simulink model "pwtsimplificado_longitudinal"  (R2025a)
settings: Solver=ode3  StartTime=0.0  StopTime=12  FixedStep=Amostragem/10  RelTol=1e-3
InitFcn:
  | % Suprime os warnings de limite do MFeval. Eles disparam A CADA PASSO quando o pneu
  | % opera fora da faixa do .tir (frenagem forte, baixa velocidade, Fz baixo) e chegam a
  | % custar 10x o tempo de simulacao. Os valores ja sao saturados internamente pelo solver.
  | warning('off','Solver:Limits:Exceeded');
  | warning('off','Solver:CoeffChecks:Ex');
model workspace (MATLAB code in the model file):
  | %% =======================================================================
  | %  INICIALIZACAO - Powertrain VE (motor de inducao Hercules AMP223/226
  | %  + SEVCON Gen5, IRFOC)  -  rev. 4 (identificacao + fix Vmag + dados AMP-226)
  | %  -----------------------------------------------------------------------
  | %  CONVENCAO: correntes/tensoes de fase em VALORES DE PICO (Park/Clarke
  | %  amplitude-invariantes). Valores RMS da folha convertidos com sqrt(2).
  | %
  | %  PARAMETROS DO MOTOR: identificados por minimos quadrados sobre as 20
  | %  linhas das tabelas do dinamometro (residuo RMS 3.3%). Modelo LINEAR,
  | %  valido na regiao de fluxo parcial (Id <= ~110 A pico) onde o modelo e
  | %  o controlador operam. Os valores de placa "133 A nominal" e "114 A a
  | %  vazio" sao pontos de fluxo pleno SATURADO - o modelo linear NAO os
  | %  reproduz e NAO deve reproduzir. NAO "corrigir" Imag de volta p/ 114*sqrt(2).
  | %
  | %  ATENCAO: o BLOCO DA MAQUINA no subsistema Motor precisa carregar estes
  | %  mesmos Lm/Lls/Llr/Rr/Rs - controlador e planta com motores diferentes
  | %  recria o descasamento que ja foi depurado.
  | %% =======================================================================
  | %% --- Acumulador (lado DC) ----------------------------------------------
  | Bi = 250 ;             % Corrente DC maxima do acumulador (A) - limite de POTENCIA no lado DC.
  |                        %   NAO usar como limite de corrente de fase (ver I_max).
  |                        %   Com 28 kW de pico e EFF ~83%: 234 A @144V -> so 6% de folga.
  | Bv = 168 ;             % Tensao do acumulador (V) - carga cheia (nominal ~144 V)
  | %% --- Motor (identificado a partir das tabelas da folha) ----------------
  | Pnom  = 11000 ;        % Potencia nominal do motor (W)
  | T_max = 94 ;           % Torque maximo/pico 2-min (N*m) - usar na saturacao de Torque_ref
  | Poles = 2 ;            % Numero de PARES de polos (motor de 4 polos -> Poles = 2)
  | Rs  = 0.0165 ;         % Resistencia do estator por fase (Ohm) - folha obs.9: 0.033 de linha /2
  |                        %   (a identificacao usou 0.0144 fixo; diferenca so mexe ~7% no Ki)
  | Rr  = 0.01858 ;        % Resistencia do rotor referida ao estator (Ohm) - IDENTIFICADO
  |                        %   NUNCA usar 0.0248/0.0139: 0.0248 veio do Tau_r=35.5ms
  |                        %   INTERMEDIARIO ERRADO (assumia Kt/Imag antigos); reverter se aparecer.
  | Lls = 7.4763e-5 ;      % Indutancia de dispersao do estator (H) - IDENTIFICADO (Lls=Llr imposto)
  | Llr = 7.4763e-5 ;      % Indutancia de dispersao do rotor (H)   - IDENTIFICADO
  | Lm  = 1.0357e-3 ;      % Indutancia de magnetizacao (H) - IDENTIFICADO (valor LINEAR, fluxo parcial)
  | Ls  = Lls + Lm ;       % Indutancia total do estator (H)  = 1.1105e-3
  | Lr  = Lm + Llr ;       % Indutancia total do rotor (H)    = 1.1105e-3
  | Im  = 0.0071 ;         % Inercia do rotor (kg*m^2). A folha escreve "kgfm2" mas o valor e SI:
  |                        %   carcaca 100 limita o rotor a r<~7cm -> J~0.007-0.01 kg*m^2;
  |                        %   0.0697 (x9.81) exigiria r~12cm, impossivel. [dica: Im=100 trava o rotor]
  | motor_eff = 0.874 ;    % Eficiencia nominal do motor (-) (folha: 87.4% nominal, ~83% no pico)
  | mc_eff    = 0.95 ;     % Eficiencia do inversor (-)
  | %% --- Constantes derivadas do motor -------------------------------------
  | sigma = 1 - (Lm^2)/(Ls*Lr) ;      % Coef. de dispersao total (-)             ~0.1301
  | Tau_r = Lr/Rr ;                   % Constante de tempo do rotor (s)          ~59.8 ms
  |                                   %   Gain "1/Tau_r" embutido no modelo -> 16.73
  | Kt    = (3/2)*Poles*(Lm^2/Lr) ;   % Constante de torque p/ correntes de PICO ~2.898e-3 N*m/A^2
  | Req   = Rs + Rr*((Lm/Lr)^2) ;     % Resistencia equivalente da malha de corrente (Ohm) ~0.0327
  | %% --- Correntes de referencia (PICO de fase) ----------------------------
  | Imag  = 105 ;          % Corrente de magnetizacao (A PICO) - IDENTIFICADA (74 A RMS).
  |                        %   NAO e a "corrente a vazio" da folha (114 RMS = fluxo pleno SATURADO,
  |                        %   fora da regiao linear). Constant "Imag" embutida no modelo -> 105.
  | Idref = Imag ;         % Referencia inicial de corrente do eixo d (A pico)
  | I_max_motor = 242*sqrt(2) ; % Pico 2-min do MOTOR (242 A RMS -> 342.2 pico) - folha
  | I_max_inv   = 257*sqrt(2) ; % Limite AC 1-min do SEVCON Gen5 (257 A RMS -> 363.5 pico)
  | I_max = min(I_max_motor, I_max_inv) ; % limite operativo = o mais restritivo (342.2 pico)
  | % Iq_sat e calculado DINAMICAMENTE no modelo: sqrt(max(I_max^2 - Idref^2, 0))
  | % (limite de corrente vetorial com prioridade ao eixo d - correto)
  | % Torque max alcancavel: Kt*Imag*sqrt(I_max^2-Imag^2) = 99.1 N*m > T_max ✓
  | %% --- Controle discreto / modulacao -------------------------------------
  | Amostragem = 1.25e-4 ; % Periodo de amostragem do controle discreto (s) - 8 kHz
  | Modulation_Target = 0.95 ; % Indice de modulacao alvo (-) - margem antes da sobremodulacao
  | Vmax = (Bv*Modulation_Target)/sqrt(3) ; % Teto de tensao de fase em pico (V)  ~92.1 V
  | % Vq_lim e calculado DINAMICAMENTE no modelo: sqrt(max(Vmax^2 - Vd_sat^2, 0))
  | % (saturacao de tensao vetorial com prioridade ao Vd - correto)
  | c_comp = 1.5 ;         % Compensacao de atraso de angulo (amostras): theta_comp = theta + We*c_comp*Amostragem
  |                        %   SO no caminho de ATUACAO (Inverse Park); a Park direta usa theta puro.
  | %% --- Malha de corrente: ganhos (base p/ parametrizar o SEVCON Gen5) ----
  | wc  = 2*pi*200 ;       % Largura de banda desejada da malha de corrente (rad/s)
  |                        %   regra: wc*Amostragem << 1  (aqui ~0.157, OK)
  | Kp  = sigma*Ls*wc ;    % Ganho proporcional (V/A)        ~0.182
  | Ki  = Req*wc ;         % Ganho integral (V/(A*s))        ~41.0
  | Kaw = Ki/Kp ;          % Anti-windup back-calculation (1/s)  ~226
  |                        %   NUNCA usar 1/(Kp*Amostragem): da Kaw*Ts ~ 2 e diverge.
  |                        %   Conferir: Kaw*Amostragem << 1 (aqui ~0.028)
  | %% --- Field weakening (PI discreto com anti-windup) ---------------------
  | wc_fw     = 2*pi*15 ;              % Banda do laco de FW (rad/s) - MUITO mais lento que wc
  | Fw_margin = 0.95 ;                 % FW age ANTES da saturacao vetorial de tensao.
  |                                    %   NAO criar essa margem baixando Modulation_Target.
  | V_ref_fw  = Vmax*Fw_margin ;       % Referencia do laco de FW (~87.5 V pico de fase)
  | We_base = 2*pi*103 ;               % Ponto de projeto = velocidade base eletrica (rad/s)
  | Kv_fw   = We_base*Ls ;             % Ganho ideal da planta Id->Vmag (~0.719 V/A)
  | Kp_fw  = (1/Kv_fw)/3 ;             % ~0.46 A/V. Margem /3 sobre o ganho ideal.
  |                                    %   HISTORICO: o /10 antigo compensava um BUG ja corrigido:
  |                                    %   a cadeia do Vmag (u^2 -> 1/z -> sqrt -> filtro) rodava na
  |                                    %   taxa do SOLVER (sample time herdado) e lia o PICO do ripple
  |                                    %   intra-amostra (+26 V). Com a cadeia em Amostragem, /3 e
  |                                    %   estavel, sem ciclo limite, e o FW nao fica lento demais.
  | Ki_fw  = Kp_fw*(wc_fw/3) ;         % ~14.6 A/(V*s)
  | Kaw_fw = Ki_fw/Kp_fw ;             % = wc_fw/3 ~ 31.4 1/s
  | Id_min_pu = 0.15 ;                 % Piso de campo (15% de Imag)
  | dImag_max = 0 ;                    % FW so REDUZ campo (saturacao superior = 0)
  | dImag_min = -(1-Id_min_pu)*Imag ;  % Saturacao inferior = -89.25 A (piso garantido AQUI;
  |                                    %   nao por outro Saturation no Id_ref)
  | f_lp_vmag = 50 ;                   % Filtro passa-baixa no V_mag ANTES do somador de erro (Hz)
  | a_vmag    = exp(-2*pi*f_lp_vmag*Amostragem) ; % 0.9615 a 8 kHz
  |                                    %   Discrete TF: [1-a_vmag] / [1 -a_vmag]
  |                                    %   ATENCAO: TODA a cadeia do Vmag (2x Unit Delay, u^2, filtro)
  |                                    %   precisa de Sample Time = Amostragem EXPLICITO nos blocos.
  |                                    %   Herdado (-1) roda na taxa do solver e le o pico do ripple.
  | assert(Kaw_fw*Amostragem < 0.1, 'Kaw_fw alto demais')
  | %% --- Transmissao / roda ------------------------------------------------
  | gear_ratio = 4.45 ;    % Relacao de transmissao (-)
  | trans_eff  = 0.89 ;    % Eficiencia da transmissao (-)
  | Rw = 0.2605 ;          % Raio da roda (m)
  | Iw = 1.20 ;            % Inercia das rodas TRACIONADAS (kg*m^2)
  | 
  | %% --- Freios (dinamica longitudinal) ------------------------------------
  | T_brake_max = 1700 ;   % Torque de freio max TOTAL nas rodas (N*m) - ESTIMADO pelo limite
  |                        %   de pneu da planilha (muf=1.8: 1.8*m*g*Rw ~ 1683). Medir o real.
  | brake_bias_f = 0.70 ;  % Fracao do freio no eixo DIANTEIRO - ESTIMADA (balance bar).
  |                        %   Aqui so o traseiro entra na Transmissao; o dianteiro vira uma
  |                        %   forca de frenagem direta no Veiculo (nao ha roda dianteira neste
  |                        %   modelo longitudinal).
  | brake_cut = 0.15 ;     % Pedal acima disso CORTA o torque do motor (brake override, como a VCU)
  | mu_scale = 1.0 ;       % Derating de pista p/ o muRoad do MFeval. O .tir da mu~2.45 (bancada);
  |                        %   a planilha do carro usa 1.7-1.8 (pista real) -> mu_scale ~0.70.
  |                        %   ATENCAO: conferir se ja soma as 2 rodas (Fx do pneu e x2 no Pneu).
  |                        %   Planilha: rodas traseiras = 22 kg o par (11 kg/roda) -> estimativa
  |                        %   ~0.45 kg*m^2/roda (~0.9 o par) + coroa/semieixos. 1.2 e plausivel;
  |                        %   vale medir/calcular no CAD.
  | %% --- Veiculo (dinamica longitudinal) - dados AMP-226 (planilha ago/2026) ---
  | m  = 366 ;             % Massa total com piloto (kg) - aba "Dados Tecnicos"
  |                        %   (a aba "Comportamento do Carro" usa 358.8; diferenca de 2%,
  |                        %    conferir com a equipe qual e a pesagem vigente)
  | g  = 9.81 ;            % Aceleracao da gravidade (m/s^2)
  | air_density = 1.225 ;  % Densidade do ar (kg/m^3)
  | Af = 1.17 ;            % Area frontal (m^2)            - aba "Acoes de aero"
  | Cd = 1.06 ;            % Coef. de arrasto (-)          - aba "Acoes de aero" (CdA = 1.24)
  | Cr = 0.02 ;            % Coef. de resistencia de rolagem (-) - aba "LoadCasesNico" (f = 0.02)
  | %% --- Geometria e cargas (p/ Fz dinamico no pneu) - dados AMP-226 -------
  | L_wb      = 1.56 ;     % Entre-eixos (m)
  | dist_cg_f = 0.804 ;    % Distancia do CG ao eixo DIANTEIRO (m)
  | frac_rear = dist_cg_f/L_wb ; % Fracao de massa no eixo traseiro = 0.5154
  | h_cg      = 0.295 ;    % Altura do CG (m) - calculada; "CG estimado" da planilha = 0.315
  | Fz_rear_static = m*g*frac_rear/2 ; % Carga estatica por roda TRASEIRA = 925.2 N
  |                        %   (Constant "Fz" no subsistema Pneu: era 889 -> usar 925.2,
  |                        %    ou melhor, o Fz dinamico abaixo)
  | ClA_total = 2.11 ;     % Area de lift total (m^2) - tabela de downforce x velocidade da
  |                        %   aba "Acoes de aero" (consistente de 60 a 110 km/h)
  | downforce_rear_share = 0.48 ; % Fracao do downforce no eixo traseiro - ATENCAO: a planilha
  |                        %   tem valores conflitantes (0.45 a 0.58 conforme a aba);
  |                        %   conferir com o subsistema de aero
  | K_transf = (m*h_cg/L_wb)/2 ;       % Ganho ax -> dFz por roda (N por m/s^2) ~34.6
  | K_downf  = 0.5*air_density*ClA_total*downforce_rear_share/2 ; % Ganho Vx^2 -> dFz por roda
  | % Fz dinamico por roda traseira - JA FIADO no subsistema Pneu:
  | %   Fz_rear = Fz_rear_static + K_transf*ax_filtrado + K_downf*Vx^2
  | %   ax vem do Goto global "ax" (saida do ganho 1/m no subsistema Veiculo),
  | %   filtrado por 1/(0.1s+1) - quebra o laco algebrico Fz->Fx->ax->Fz e representa
  | %   a dinamica da suspensao na transferencia de carga.
  | %% --- Condicoes iniciais dos sinais -------------------------------------
  | % Evitam divisao por zero no controlador e singularidade de escorregamento
  | % do modelo de pneu (MFeval) em Vx = 0.
  | Velocity    = 0.1 ;    % Velocidade inicial do veiculo (m/s)
  | Wheel_Speed = 1 ;      % Velocidade angular inicial da roda (rad/s)
  | Iqref = 0.1 ;          % Valor inicial da referencia de corrente do eixo q (A)
  | Vd    = 0.1 ;          % Valor inicial da tensao do eixo d (V)
  | Vq    = 0.1 ;          % Valor inicial da tensao do eixo q (V)
  | %% --- Pneu (MFeval) -----------------------------------------------------
  | % Arquivo .tir procurado a partir da pasta do modelo (data/ ou ao lado do .slx),
  | % depois no path do MATLAB - nada de caminho absoluto, roda em qualquer maquina.
  | tirNome = 'Avon_9760_Round_2.tir';
  | try, raizModelo = fileparts(get_param('pwtsimplificado_longitudinal','FileName')); catch, raizModelo = pwd; end
  | tirFile = '';
  | for c = {fullfile(raizModelo,'data',tirNome), fullfile(raizModelo,tirNome), which(tirNome)}
  |     if ~isempty(c{1}) && isfile(c{1}), tirFile = c{1}; break, end
  | end
  | assert(~isempty(tirFile), 'Arquivo %s nao encontrado em %s/data nem no path do MATLAB.', tirNome, raizModelo);
  | tirParams = mfeval.readTIR(tirFile);
  | %% --- Verificacoes rapidas (rodar sempre que mudar parametros) ----------
  | fprintf('--- Verificacoes ---\n');
  | fprintf('Kaw*Ts   = %.4f | wc*Ts = %.4f  (ambos << 1)\n', Kaw*Amostragem, wc*Amostragem);
  | fprintf('sigma    = %.4f (esperado 0.130) | Tau_r = %.1f ms (esperado 59.8 - se der ~35, Rr esta ERRADO)\n', sigma, Tau_r*1e3);
  | fprintf('Kt = %.4g (esperado 2.898e-3) | Req = %.4g\n', Kt, Req);
  | fprintf('Kp = %.3f V/A | Ki = %.1f V/(A*s) | Kaw = %.1f 1/s\n', Kp, Ki, Kaw);
  | fprintf('FW: Kp_fw = %.3f | Ki_fw = %.2f | Kaw_fw = %.2f | dImag_min = %.2f\n', Kp_fw, Ki_fw, Kaw_fw, dImag_min);
  | fprintf('Vmax = %.1f V | V_ref_fw = %.1f V | Imag = %.0f A pico | I_max = %.1f A pico\n', Vmax, V_ref_fw, Imag, I_max);
  | fprintf('Torque max alcancavel = %.1f N*m (deve ser > T_max = %.0f)\n', Kt*Imag*sqrt(I_max^2-Imag^2), T_max);
  | fprintf('--- Alvos de aceitacao (tabelas da folha, NAO o cabecalho) ---\n');
  | Iq35 = 35/(Kt*Imag); Iq94 = 94/(Kt*Imag);
  | fprintf('35 N*m: I = %.1f A RMS (folha sub-base: 110-111) | slip = %.2f Hz (folha: 3.0-3.3)\n', ...
  |         sqrt(Imag^2+Iq35^2)/sqrt(2), Iq35/(Tau_r*Imag)/(2*pi));
  | fprintf('94 N*m: I = %.1f A RMS (folha: 240; ~4%% de folga = saturacao/ferro) | slip = %.2f Hz (folha: ~8)\n', ...
  |         sqrt(Imag^2+Iq94^2)/sqrt(2), Iq94/(Tau_r*Imag)/(2*pi));
  | fprintf('Joelho de FW esperado: ~2970 RPM a torque pleno | Id_ref >= %.0f A ate 4800 RPM\n', 0.55*Imag);
  | fprintf('P_DC: disponivel %.1f kW | pico estimado %.1f kW (com EFF pico 0.83)\n', Bv*Bi/1e3, 28/0.83);
undefined symbols (not defined in the file): DiscIntNeverNeededParam, dspblkCoreblockFVToolHelper, gcbh, sigbuilder_block, Vq_lim
libraries: mcbeeMathTransformLib x4, spsControlledVoltageSourceLib x3, spsGroundLib x3, simulink x2, spsAsynchronousMachineSIUnitsLib x1, spspowerguiLib x1, mfeval_LIB x1
settings Model: Creator=gabox  LastModifiedBy=gabox
settings ModelReferenceCC: EnableRefExpFcnMdlSchedulingChecks=on
settings RTWCC: GPUComputeCapability=3.5

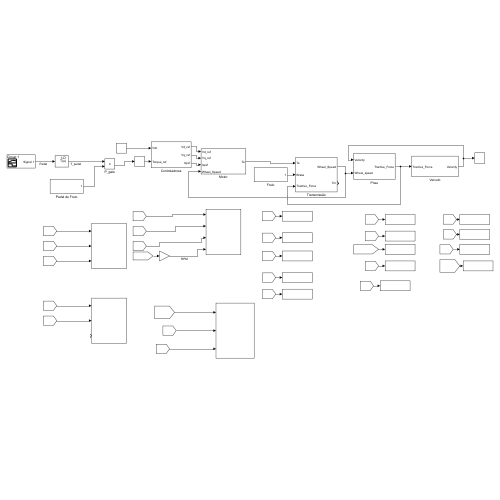
[thumbnail: Simulink's stored preview of the top-level diagram]
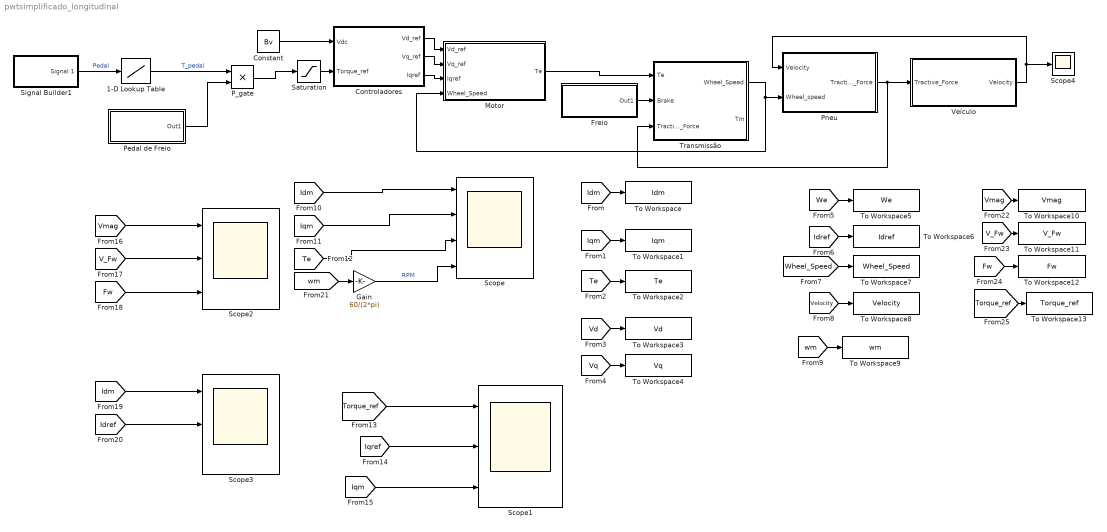
== system pwtsimplificado_longitudinal ==
  1-D Lookup Table : Lookup_n-D  NumberOfTableDimensions=1  BreakpointsForDimension1=[0 T_max]  Table=[0 T_max]  InternalRulePriority=Speed  RndMeth=Simplest
  Constant : Constant  Value=Bv
  Controladores : Subsystem
  Freio : Subsystem
  Gain : Gain  Gain=60/(2*pi)
  Motor : Subsystem
  P_gate : Product
  Pedal de Freio : Subsystem
  Pneu : Subsystem
  Saturation : Saturate  UpperLimit=T_max  LowerLimit=0
  Scope : Scope  NumInputPorts=4
      settings: ActiveDisplayYMinimum=-590.16438229728544  ActiveDisplayYMaximum=5311.47944067557  DataLoggingVariableName=ScopeData2
  Scope1 : Scope  NumInputPorts=3
      settings: ActiveDisplayYMinimum=-42.119926332695584  ActiveDisplayYMaximum=379.0793369942603  DataLoggingVariableName=ScopeData3
  Scope2 : Scope  NumInputPorts=3
      settings: ActiveDisplayYMinimum=-173.12729270620673  ActiveDisplayYMaximum=187.77269241633141  DataLoggingVariableName=ScopeData4
  Scope3 : Scope  NumInputPorts=3
      settings: ActiveDisplayYMinimum=-22.382704849224424  ActiveDisplayYMaximum=201.44434364301986
  Scope4 : Scope
      settings: DataLoggingVariableName=ScopeData5
  Signal Builder1 : Subsystem  Tag=STV Subsys  LoadFcn=sigbuilder_block('load');  StartFcn=sigbuilder_block('start');  StopFcn=sigbuilder_block('stop');  ClipboardFcn=sigbuilder_block('clipboard');  mask(Sigbuilder block){tuvar=[0:10]}
      mask help: Simulink:masks:SigbuilderBlock_MD
      mask init:
      | if ~strcmp(get_param(bdroot(gcbh),'SimulationStatus'),'stopped') tuvar = sigbuilder_block('maskInit'); end
      settings: CopyFcn=sigbuilder_block('copy');  DeleteFcn=sigbuilder_block('delete');  ModelCloseFcn=sigbuilder_block('modelClose');  PreSaveFcn=sigbuilder_block('preSave');  PauseFcn=sigbuilder_block('pause');  ContinueFcn=sigbuilder_block('continue');  NameChangeFcn=sigbuilder_block('namechange');  OpenFcn=sigbuilder_block('open',[252.75 107.25 644.25 387.75 ]);  CloseFcn=sigbuilder_block('close');
      mask Display: plot(0, 0, 100, 100,[2, 2, 32, 32, 2], [68, 8, 8, 68, 68],[32, 2], [38, 38], [32, 19, 2],[53, 60, 44], [32, 17, 17, 2],[16, 16, 31, 31]);txt = getActiveGroup(gcbh);text(2, 100, txt,'verticalAlignment', 'top');
  To Workspace : ToWorkspace  VariableName=Idm  SaveFormat=Timeseries  SampleTime=Amostragem
  To Workspace1 : ToWorkspace  VariableName=Iqm  SaveFormat=Timeseries  SampleTime=Amostragem
  To Workspace10 : ToWorkspace  VariableName=Vmag  SaveFormat=Timeseries  SampleTime=Amostragem
  To Workspace11 : ToWorkspace  VariableName=V_Fw  SaveFormat=Timeseries  SampleTime=Amostragem
  To Workspace12 : ToWorkspace  VariableName=Fw  SaveFormat=Timeseries  SampleTime=Amostragem
  To Workspace13 : ToWorkspace  VariableName=Torque_ref  SaveFormat=Timeseries  SampleTime=Amostragem
  To Workspace2 : ToWorkspace  VariableName=Te  SaveFormat=Timeseries  SampleTime=Amostragem
  To Workspace3 : ToWorkspace  VariableName=Vd  SaveFormat=Timeseries  SampleTime=Amostragem
  To Workspace4 : ToWorkspace  VariableName=Vq  SaveFormat=Timeseries  SampleTime=Amostragem
  To Workspace5 : ToWorkspace  VariableName=We  SaveFormat=Timeseries  SampleTime=Amostragem
  To Workspace6 : ToWorkspace  VariableName=Idref  SaveFormat=Timeseries  SampleTime=Amostragem
  To Workspace7 : ToWorkspace  VariableName=Wheel_Speed  SaveFormat=Timeseries  SampleTime=Amostragem
  To Workspace8 : ToWorkspace  VariableName=Velocity  SaveFormat=Timeseries  SampleTime=Amostragem
  To Workspace9 : ToWorkspace  VariableName=wm  SaveFormat=Timeseries  SampleTime=Amostragem
  Transmissão : Subsystem
  Veículo : Subsystem
  wires:
  Transmissão/1(Wheel_Speed) -> Pneu/2(Wheel_speed), Motor/4(Wheel_Speed)
  Veículo/1(Velocity) -> Pneu/1(Velocity), Scope4/1
  Motor/1(Te) -> Transmissão/1(Te)
  Pneu/1(Tractive_Force) -> Transmissão/3(Tractive_Force), Veículo/1(Tractive_Force)
  Controladores/1(Vd_ref) -> Motor/1(Vd_ref)
  Controladores/2(Vq_ref) -> Motor/2(Vq_ref)
  Constant/1 -> Controladores/1(Vdc)
  Saturation/1 -> Controladores/2(Torque_ref)
  Controladores/3(Iqref) -> Motor/3(Iqref)
  Signal Builder1/1(Signal 1) -> 1-D Lookup Table/1  "Pedal"
  [Idm] -> To Workspace/1
  [Iqm] -> To Workspace1/1
  [Vd] -> To Workspace3/1
  [Te] -> To Workspace2/1
  [Vq] -> To Workspace4/1
  [Idref] -> To Workspace6/1
  [We] -> To Workspace5/1
  [Wheel_Speed] -> To Workspace7/1
  [Velocity] -> To Workspace8/1
  [wm] -> To Workspace9/1
  [Idm] -> Scope/1
  [Iqm] -> Scope/2
  [Te] -> Scope/3
  [Torque_ref] -> Scope1/1
  [Iqref] -> Scope1/2
  [Iqm] -> Scope1/3
  [Fw] -> Scope2/3
  [Vmag] -> Scope2/1
  [V_Fw] -> Scope2/2
  [Idm] -> Scope3/1
  [Idref] -> Scope3/2
  [wm] -> Gain/1
  [Vmag] -> To Workspace10/1
  [V_Fw] -> To Workspace11/1
  [Fw] -> To Workspace12/1
  [Torque_ref] -> To Workspace13/1
  Gain/1 -> Scope/4  "RPM"
  1-D Lookup Table/1 -> P_gate/1  "T_pedal"
  P_gate/1 -> Saturation/1
  Freio/1(Out1) -> Transmissão/2(Brake)
  Pedal de Freio/1(Out1) -> P_gate/2

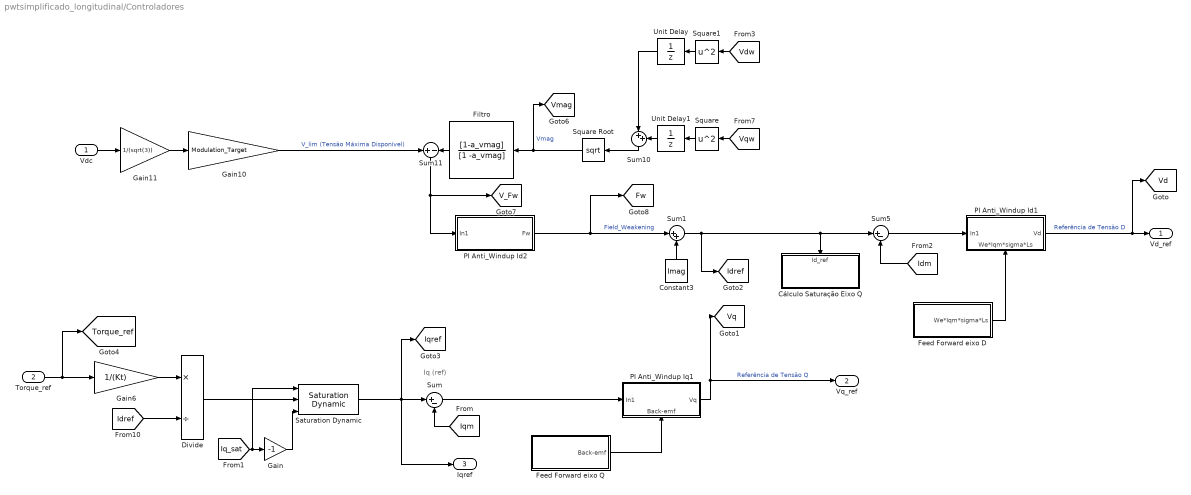
== system pwtsimplificado_longitudinal/Controladores ==
  note: Iq (ref)
  Vdc : Inport
  Torque_ref : Inport  Port=2
  Constant3 : Constant  Value=Imag
  Cálculo Saturação Eixo Q : Subsystem
      settings: PortSchema="{\"entries\":[{\"content\":{\"sides\":[{\"content\":{},\"type\":\"ConnectorPlacement.EquallySpacedRectSide\",\"uuid\":\"7f7fb8a8-2f6b-4961-9c00-1f4e2fc5b775\"},{\"content\":{\"side\":\"RIGHT\"},\"type\":\"ConnectorPlacement.EquallySpacedRectSide\",\"uuid\":\"99257d35-6f07-42ed-a793-bbf32f624519\"},{\"content\":{\"connectorIds\":[\"In1\"],\"side\":\"TOP\"},\"type\":\"ConnectorPlacement.EquallySpacedRectSide\",\"uuid\":\"78fef148-479c-4404-810b-4f212cfc0a7c\"}]},\"type\":\"ConnectorPlacement.EquallySpacedConnector\",\"uuid\":\"0774de6e-bcfc-41a2-9f60-6d7989875326\"}],\"packageUris\":[\"http://schema.mathworks.com/mf0/Connector/R2020b\"],\"version\":\"1.0\"}"
  Divide : Product  Inputs=*/
  Feed Forward eixo D : Subsystem
  Feed Forward eixo Q : Subsystem
  Filtro : DiscreteTransferFcn  LoadFcn=dspblkCoreblockFVToolHelper(gcbh,'load');  Numerator=[1-a_vmag]  Denominator=[1 -a_vmag]  SampleTime=Amostragem
      settings: CopyFcn=dspblkCoreblockFVToolHelper(gcbh,'copy');  DeleteFcn=dspblkCoreblockFVToolHelper(gcbh,'close');  ModelCloseFcn=dspblkCoreblockFVToolHelper(gcbh,'close');  PreSaveFcn=dspblkCoreblockFVToolHelper(gcbh,'presave');  PostSaveFcn=dspblkCoreblockFVToolHelper(gcbh,'postsave');  CloseFcn=dspblkCoreblockFVToolHelper(gcbh,'close');
  Gain : Gain  Gain=-1
  Gain10 : Gain  Gain=Modulation_Target
  Gain11 : Gain  Gain=1/(sqrt(3))
  Gain6 : Gain  Gain=1/(Kt)
  PI Anti_Windup Id1 : Subsystem
      settings: PortSchema="{\"entries\":[{\"content\":{\"sides\":[{\"content\":{\"connectorIds\":[\"In1\"]},\"type\":\"ConnectorPlacement.EquallySpacedRectSide\",\"uuid\":\"0de77585-2e0a-4dcb-a42d-23ce97468db2\"},{\"content\":{\"connectorIds\":[\"Out1\"],\"side\":\"RIGHT\"},\"type\":\"ConnectorPlacement.EquallySpacedRectSide\",\"uuid\":\"33b7113f-9ed7-41a2-ab15-fe3179c74bc1\"},{\"content\":{\"connectorIds\":[],\"side\":\"TOP\"},\"type\":\"ConnectorPlacement.EquallySpacedRectSide\",\"uuid\":\"80085514-688f-4280-b0ee-d4b30b84859c\"},{\"content\":{\"connectorIds\":[\"In2\"],\"side\":\"BOTTOM\"},\"type\":\"ConnectorPlacement.EquallySpacedRectSide\",\"uuid\":\"df22b881-1b5e-45ae-891f-eebf20510deb\"}]},\"type\":\"ConnectorPlacement.EquallySpacedConnector\",\"uuid\":\"87582b80-d1ad-469a-97fa-00e7f61ced2e\"}],\"packageUris\":[\"http://schema.mathworks.com/mf0/Connector/R2020b\"],\"version\":\"1.0\"}"
  PI Anti_Windup Id2 : Subsystem
  PI Anti_Windup Iq1 : Subsystem
      settings: PortSchema="{\"entries\":[{\"content\":{\"sides\":[{\"content\":{\"connectorIds\":[\"In1\"]},\"type\":\"ConnectorPlacement.EquallySpacedRectSide\",\"uuid\":\"0de77585-2e0a-4dcb-a42d-23ce97468db2\"},{\"content\":{\"connectorIds\":[\"Out1\"],\"side\":\"RIGHT\"},\"type\":\"ConnectorPlacement.EquallySpacedRectSide\",\"uuid\":\"33b7113f-9ed7-41a2-ab15-fe3179c74bc1\"},{\"content\":{\"connectorIds\":[],\"side\":\"TOP\"},\"type\":\"ConnectorPlacement.EquallySpacedRectSide\",\"uuid\":\"80085514-688f-4280-b0ee-d4b30b84859c\"},{\"content\":{\"connectorIds\":[\"In2\"],\"side\":\"BOTTOM\"},\"type\":\"ConnectorPlacement.EquallySpacedRectSide\",\"uuid\":\"df22b881-1b5e-45ae-891f-eebf20510deb\"}]},\"type\":\"ConnectorPlacement.EquallySpacedConnector\",\"uuid\":\"87582b80-d1ad-469a-97fa-00e7f61ced2e\"}],\"packageUris\":[\"http://schema.mathworks.com/mf0/Connector/R2020b\"],\"version\":\"1.0\"}"
  Saturation Dynamic : simulink/Discontinuities/Saturation Dynamic  OutMin=[]  OutMax=[]  OutDataTypeStr=Inherit: Same as second input  OutDataType=fixdt(1, 16)  OutScaling=2^-10  DoSatur=off
  Square : Math  Operator=square
  Square Root : Sqrt
  Square1 : Math  Operator=square
  Sum : Sum  Inputs=|+-
  Sum1 : Sum  Inputs=|++
  Sum10 : Sum  Inputs=|++
  Sum11 : Sum  Inputs=+|-
  Sum5 : Sum  Inputs=|+-
  Unit Delay : UnitDelay  SampleTime=Amostragem  HasFrameUpgradeWarning=on
  Unit Delay1 : UnitDelay  SampleTime=Amostragem  HasFrameUpgradeWarning=on
  Vd_ref : Outport
  Vq_ref : Outport  Port=2
  Iqref : Outport  Port=3
  tag scope: Fw=global, Idref=global, Iqref=global, Torque_ref=global, V_Fw=global, Vd=global, Vmag=global, Vq=global
  wires:
  PI Anti_Windup Id2/1(Fw) -> [Fw], Sum1/1  "Field_Weakening"
  Vdc/1 -> Gain11/1
  Sum5/1 -> PI Anti_Windup Id1/1(In1)
  Sum11/1 -> [V_Fw], PI Anti_Windup Id2/1(In1)
  Gain11/1 -> Gain10/1
  Sum/1 -> PI Anti_Windup Iq1/1(In1)
  PI Anti_Windup Iq1/1(Vq) -> Vq_ref/1, [Vq]  "Referência de Tensão Q"
  Gain10/1 -> Sum11/1  "V_lim (Tensão Máxima Disponível)"
  [Idm] -> Sum5/2
  PI Anti_Windup Id1/1(Vd) -> [Vd], Vd_ref/1  "Referência de Tensão D"
  Square Root/1 -> Filtro/1, [Vmag]  "Vmag"
  Constant3/1 -> Sum1/2
  Sum1/1 -> Sum5/1, Cálculo Saturação Eixo Q/1(Id_ref), [Idref]
  Sum10/1 -> Square Root/1
  Unit Delay1/1 -> Sum10/2
  Unit Delay/1 -> Sum10/1
  Square/1 -> Unit Delay1/1
  Square1/1 -> Unit Delay/1
  [Iqm] -> Sum/2
  Torque_ref/1 -> [Torque_ref], Gain6/1
  [Idref] -> Divide/2
  Gain6/1 -> Divide/1
  Feed Forward eixo D/1(We*Iqm*sigma*Ls) -> PI Anti_Windup Id1/2(We*Iqm*sigma*Ls)
  Feed Forward eixo Q/1(Back-emf) -> PI Anti_Windup Iq1/2(Back-emf)
  Divide/1 -> Saturation Dynamic/2
  Saturation Dynamic/1 -> [Iqref], Iqref/1, Sum/1
  [Iq_sat] -> Saturation Dynamic/1, Gain/1
  Gain/1 -> Saturation Dynamic/3
  [Vdw] -> Square1/1
  [Vqw] -> Square/1
  Filtro/1 -> Sum11/2

== system pwtsimplificado_longitudinal/Freio ==
  G_Tbr : Gain  Gain=(1-brake_bias_f)*T_brake_max
  P_Tbr : Product
  Tanh_wr : Trigonometry  Operator=tanh
  Out1 : Outport
  wires:
  [Brake_pedal] -> G_Tbr/1
  [Wheel_Speed] -> Tanh_wr/1
  Tanh_wr/1 -> P_Tbr/2
  G_Tbr/1 -> P_Tbr/1
  P_Tbr/1 -> Out1/1

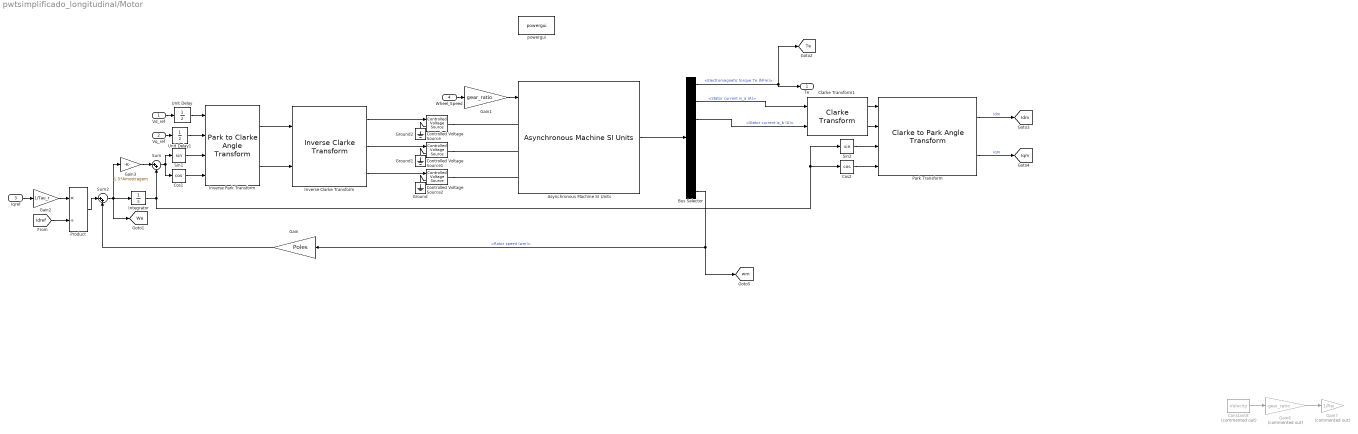
== system pwtsimplificado_longitudinal/Motor ==
  Vd_ref : Inport
  Vq_ref : Inport  Port=2
  Iqref : Inport  Port=3
  Wheel_Speed : Inport  Port=4
  Asynchronous Machine SI Units : spsAsynchronousMachineSIUnitsLib/Asynchronous Machine SI Units  RotorType=Squirrel-cage  PresetModel=No  MechanicalLoad=Speed w  ShowDetailedParameters=on  ReferenceFrame=Stationary  Units=SI  MeasurementBus=off  NominalParameters=[20143, 102, 100]  VoltageRatio=1  Stator=[Rs Lls]  Rotor=[Rr Llr]  Cage1=[0.4155 0.002066]  Cage2=[0.4168 0.0003495]  Lm=Lm  Mechanical=[Im 0.00001 Poles]  PolePairs=2  InitialConditions=[0 0 0 0 0 0 0 0]  SimulateSaturation=off  Saturation=[14.03593122, 27.81365428, 53.79336849, 72.68890987, 97.98006896, 148.6815601, 215.7428561, 302.9841135, 428.7778367 ; 230, 322, 414, 460, 506, 552, 598, 644, 690]  LoadFlowParameters=1492000  TsPowergui=0  TsBlock=Amostragem  IterativeModel=Trapezoidal non iterative  IterativeDiscreteModel=Trapezoidal non iterative  Pmec=Pnom
  Bus Selector : BusSelector  OutputSignals=Mechanical.Electromagnetic torque Te (N*m),Stator measurements.Stator current is_a (A),Stator measurements.Stator current is_b (A),Mechanical.Rotor angle thetam (rad),Rotor measurements.Rotor flux phir_q (V s),Rotor measurements.Rotor flux phir_d (V s),Mechanical.Rotor speed (wm)
  Clarke Transform1 : mcbeeMathTransformLib/Clarke Transform  VariantControl=Variant2  PowerInvariant=off  UseWithEmbedded=on  PhaseInput=Two inputs
      settings: LibrarySourceBlock=mcbcontrolslib/Clarke Transform
  Constant8 : Constant  Commented=on  Value=Velocity
  Controlled Voltage Source : spsControlledVoltageSourceLib/Controlled Voltage Source  Initialize=on  Source_Type=AC  Amplitude=0  Phase=0  Frequency=0  Measurements=None
  Controlled Voltage Source1 : spsControlledVoltageSourceLib/Controlled Voltage Source  Initialize=on  Source_Type=AC  Amplitude=0  Phase=0  Frequency=0  Measurements=None
  Controlled Voltage Source2 : spsControlledVoltageSourceLib/Controlled Voltage Source  Initialize=on  Source_Type=AC  Amplitude=0  Phase=0  Frequency=0  Measurements=None
  Cos1 : Trigonometry  Operator=cos
  Cos2 : Trigonometry  Operator=cos
  Gain : Gain  Gain=Poles
  Gain1 : Gain  Gain=gear_ratio
  Gain2 : Gain  Gain=1/Tau_r
  Gain3 : Gain  Gain=1.5*Amostragem
  Gain6 : Gain  Commented=on  Gain=gear_ratio
  Gain7 : Gain  Commented=on  Gain=1/Rw
  Ground : spsGroundLib/Ground  LConnTagsString=a
  Ground1 : spsGroundLib/Ground  LConnTagsString=a
  Ground2 : spsGroundLib/Ground  LConnTagsString=a
  Integrator : Integrator  WrapState=on  WrappedStateUpperValue=2*pi  WrappedStateLowerValue=0
  Inverse Clarke Transform : mcbeeMathTransformLib/Inverse Clarke Transform  PowerInvariant=off  UseWithEmbedded=on  PhaseInput=Two inputs
      settings: LibrarySourceBlock=mcbcontrolslib/Inverse Clarke Transform
  Inverse Park Transform : mcbeeMathTransformLib/Park to Clarke Angle Transform  AxisAlignment=D-axis  UseWithEmbedded=on  PhaseInput=Two inputs  ThetaInput=Sine and Cosine electrical position  AngleInput=Per-unit  N_points=1024
      settings: LibrarySourceBlock=mcbcontrolslib/Inverse Park Transform
  Park Transform : mcbeeMathTransformLib/Clarke to Park Angle Transform  AxisAlignment=D-axis  UseWithEmbedded=on  PhaseInput=Two inputs  ThetaInput=Sine and Cosine electrical position  AngleInput=Per-unit  N_points=1024
      settings: LibrarySourceBlock=mcbcontrolslib/Park Transform
  Product : Product  Inputs=*/
  Sin1 : Trigonometry
  Sin2 : Trigonometry
  Sum : Sum  Inputs=|++
  Sum2 : Sum  Inputs=|++
  Unit Delay : UnitDelay  SampleTime=Amostragem  HasFrameUpgradeWarning=on
  Unit Delay1 : UnitDelay  SampleTime=Amostragem  HasFrameUpgradeWarning=on
  powergui : spspowerguiLib/powergui  Priority=1  SimulationMode=Discrete  SampleTime=Amostragem  frequency=60  Iterations=50  frequencyindice=0  Pbase=100e6  ErrMax=1e-4  UnitsV=kV  UnitsW=MW  buscounter=0  FunctionMessages=off  echomessages=off  EnableUseOfTLC=off  CurrentSourceSwitches=off  DisableSnubberDevices=off  DisableRonSwitches=off  DisableVfSwitches=off  DisplayEquations=off  AutomaticDiscreteSolvers=off  SolverType=Tustin/Backward Euler (TBE)  Interpol=off  ExternalGateDelay=off  methode=off  Ts=100  x0status=blocks  SPID=on  SwTol=0  HookPort=off  NonlinearTolerance=1e-4  nMaxIteration=100  ContinueOnMaxIteration=off  RestoreLinks=warning  ResistiveCurrentMeasurement=off  Frange=[0:2:500]  Ylog=off  Xlog=on  ShowGrid=off  save=off  variable=ZData  structure=0  ZoomFFT=off  StartTime=0.0  cycles=1  DisplayStyle=1  fundamental=60  FreqAxis=off  MaxFrequency=1000  frequencyindicesteady=1  RmsSteady=1  display=off
  Te : Outport
  tag scope: Idm=global, Iqm=global, Te=global, We=global, wm=global
  wires:
  Inverse Park Transform/1 -> Inverse Clarke Transform/1
  Inverse Park Transform/2 -> Inverse Clarke Transform/2
  Asynchronous Machine SI Units/1 -> Bus Selector/1
  Bus Selector/1 -> Te/1, [Te]  "<Electromagnetic torque Te (N*m)>"
  Clarke Transform1/2 -> Park Transform/2
  Clarke Transform1/1 -> Park Transform/1
  Bus Selector/2 -> Clarke Transform1/1  "<Stator current is_a (A)>"
  Bus Selector/3 -> Clarke Transform1/2  "<Stator current is_b (A)>"
  Integrator/1 -> Sin2/1, Cos2/1, Sum/2
  Park Transform/1 -> [Idm]  "Idm"
  Park Transform/2 -> [Iqm]  "Iqm"
  Inverse Clarke Transform/2 -> Controlled Voltage Source1/1
  Inverse Clarke Transform/3 -> Controlled Voltage Source2/1
  Iqref/1 -> Gain2/1
  Gain2/1 -> Product/1
  Product/1 -> Sum2/1
  Gain6/1 -> Gain7/1
  Constant8/1 -> Gain6/1
  Sum2/1 -> Integrator/1, [We], Gain3/1
  Inverse Clarke Transform/1 -> Controlled Voltage Source/1
  Bus Selector/7 -> [wm], Gain/1  "<Rotor speed (wm)>"
  Unit Delay/1 -> Inverse Park Transform/1
  Unit Delay1/1 -> Inverse Park Transform/2
  [Idref] -> Product/2
  Vq_ref/1 -> Unit Delay1/1
  Vd_ref/1 -> Unit Delay/1
  Gain/1 -> Sum2/2
  Wheel_Speed/1 -> Gain1/1
  Gain1/1 -> Asynchronous Machine SI Units/1
  Cos1/1 -> Inverse Park Transform/4
  Sin1/1 -> Inverse Park Transform/3
  Gain3/1 -> Sum/1
  Sum/1 -> Cos1/1, Sin1/1
  Sin2/1 -> Park Transform/3
  Cos2/1 -> Park Transform/4
  connections:
  Controlled Voltage Source/RConn1 -- Asynchronous Machine SI Units/LConn1
  Controlled Voltage Source1/RConn1 -- Asynchronous Machine SI Units/LConn2
  Controlled Voltage Source2/RConn1 -- Asynchronous Machine SI Units/LConn3
  Ground/LConn1 -- Controlled Voltage Source2/LConn1
  Ground1/LConn1 -- Controlled Voltage Source1/LConn1
  Ground2/LConn1 -- Controlled Voltage Source/LConn1

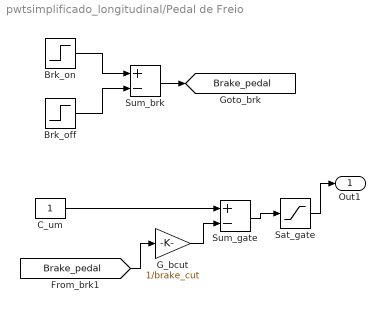
== system pwtsimplificado_longitudinal/Pedal de Freio ==
  Brk_off : Step  Time=11.5  After=0.6  SampleTime=0
  Brk_on : Step  Time=9.5  After=0.6  SampleTime=0
  C_um : Constant
  G_bcut : Gain  Gain=1/brake_cut
  Sat_gate : Saturate  UpperLimit=1  LowerLimit=0
  Sum_brk : Sum  Inputs=+-
  Sum_gate : Sum  Inputs=+-
  Out1 : Outport
  tag scope: Brake_pedal=global
  wires:
  C_um/1 -> Sum_gate/1
  [Brake_pedal] -> G_bcut/1
  Sum_gate/1 -> Sat_gate/1
  Sat_gate/1 -> Out1/1
  G_bcut/1 -> Sum_gate/2
  Brk_off/1 -> Sum_brk/2
  Sum_brk/1 -> [Brake_pedal]
  Brk_on/1 -> Sum_brk/1

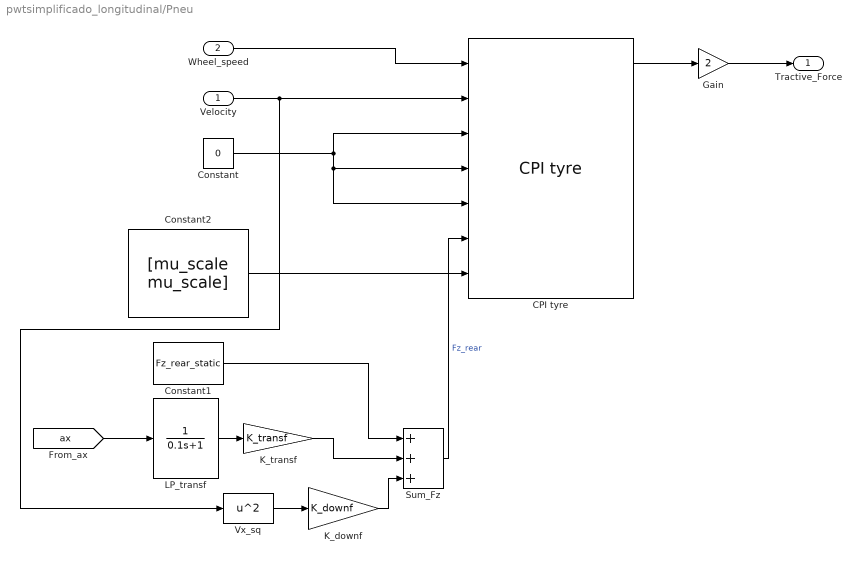
== system pwtsimplificado_longitudinal/Pneu ==
  Velocity : Inport
  Wheel_speed : Inport  Port=2
  CPI tyre : mfeval_LIB/CPI tyre  Description=Magic Formula 6.1.2 tyre model including relaxation length and transient calculations  userParameterSource=tirParams  userSide=1 left  userDynamics=1 steady state  userUseMode=1 combined  enablePressure=off  userPressure=2.3
      settings: SourceProductName=MFeval Library
  Constant : Constant  Value=0
  Constant1 : Constant  Value=Fz_rear_static
  Constant2 : Constant  Value=[mu_scale mu_scale]
  Gain : Gain  Gain=2
  K_downf : Gain  Gain=K_downf
  K_transf : Gain  Gain=K_transf
  LP_transf : TransferFcn  Denominator=[0.1 1]
  Sum_Fz : Sum  Inputs=+++
  Vx_sq : Math  Operator=square
  Tractive_Force : Outport
  wires:
  Constant/1 -> CPI tyre/5, CPI tyre/4, CPI tyre/3
  Constant2/1 -> CPI tyre/7
  CPI tyre/1 -> Gain/1
  Velocity/1 -> CPI tyre/2, Vx_sq/1
  Wheel_speed/1 -> CPI tyre/1
  Gain/1 -> Tractive_Force/1
  Constant1/1 -> Sum_Fz/1
  K_transf/1 -> Sum_Fz/2
  Vx_sq/1 -> K_downf/1
  K_downf/1 -> Sum_Fz/3
  Sum_Fz/1 -> CPI tyre/6  "Fz_rear"
  [ax] -> LP_transf/1
  LP_transf/1 -> K_transf/1

== system pwtsimplificado_longitudinal/Signal Builder1 ==
  Demux : Demux  Tag=STV Demux  Outputs=1
      settings: DisplayOption=none
  FromWs : FromWorkspace  Tag=STV FromWs  VariableName=tuvar
      SigBuilderData=|
      | common.afterFinalStr = 'Extrapolate'
      | common.sampleTime = 0
      | dataSet.timeRange = [0 10]
      | dataSet.name = 'Group 1'
      | sbobj.Groups.Name = 'Group 1'
      | sbobj.Groups.Signals.Name = 'Signal 1'
      | sbobj.Groups.Signals.XData = [0 0.1 10]
      | sbobj.Groups.Signals.YData = [0.5 100 100]
  Signal 1 : Outport  Tag=STV Outport
  wires:
  Demux/1 -> Signal 1/1
  FromWs/1 -> Demux/1

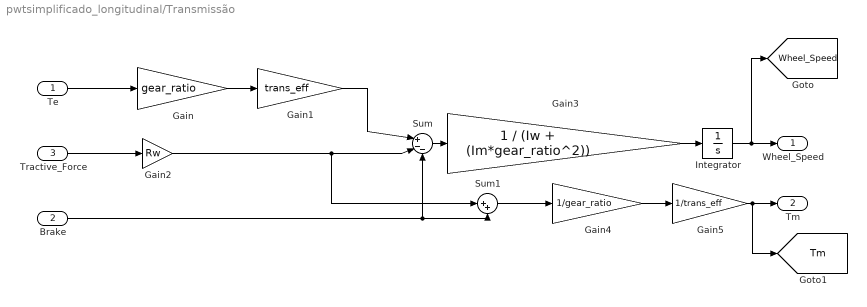
== system pwtsimplificado_longitudinal/Transmissão ==
  Te : Inport
  Brake : Inport  Port=2
  Tractive_Force : Inport  Port=3
  Gain : Gain  Gain=gear_ratio
  Gain1 : Gain  Gain=trans_eff
  Gain2 : Gain  Gain=Rw
  Gain3 : Gain  Gain=1 / (Iw + (Im*gear_ratio^2))
  Gain4 : Gain  Gain=1/gear_ratio
  Gain5 : Gain  Gain=1/trans_eff
  Integrator : Integrator
  Sum : Sum  Inputs=|+--
  Sum1 : Sum  Inputs=|++
  Wheel_Speed : Outport
  Tm : Outport  Port=2
  tag scope: Tm=global, Wheel_Speed=global
  wires:
  Gain/1 -> Gain1/1
  Tractive_Force/1 -> Gain2/1
  Gain1/1 -> Sum/1
  Gain2/1 -> Sum/2, Sum1/1
  Gain3/1 -> Integrator/1
  Sum/1 -> Gain3/1
  Brake/1 -> Sum1/2, Sum/3
  Integrator/1 -> [Wheel_Speed], Wheel_Speed/1
  Gain4/1 -> Gain5/1
  Sum1/1 -> Gain4/1
  Gain5/1 -> [Tm], Tm/1
  Te/1 -> Gain/1

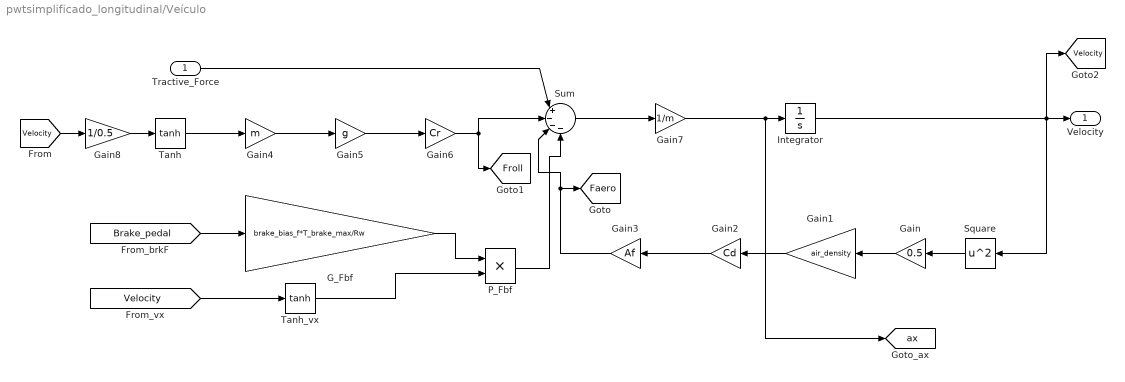
== system pwtsimplificado_longitudinal/Veículo ==
  Tractive_Force : Inport
  G_Fbf : Gain  Gain=brake_bias_f*T_brake_max/Rw
  Gain : Gain  Gain=0.5
  Gain1 : Gain  Gain=air_density
  Gain2 : Gain  Gain=Cd
  Gain3 : Gain  Gain=Af
  Gain4 : Gain  Gain=m
  Gain5 : Gain  Gain=g
  Gain6 : Gain  Gain=Cr
  Gain7 : Gain  Gain=1/m
  Gain8 : Gain  Gain=1/0.5
  Integrator : Integrator
  P_Fbf : Product
  Square : Math  Operator=square
  Sum : Sum  Inputs=|+---
  Tanh : Trigonometry  Operator=tanh
  Tanh_vx : Trigonometry  Operator=tanh
  Velocity : Outport
  tag scope: Faero=global, Froll=global, Velocity=global, ax=global
  wires:
  Integrator/1 -> [Velocity], Square/1, Velocity/1
  Gain5/1 -> Gain6/1
  Gain4/1 -> Gain5/1
  Tanh/1 -> Gain4/1
  Gain2/1 -> Gain3/1
  Gain1/1 -> Gain2/1
  Gain/1 -> Gain1/1
  Square/1 -> Gain/1
  Tractive_Force/1 -> Sum/1
  Gain6/1 -> [Froll], Sum/2
  Gain3/1 -> [Faero], Sum/3
  Sum/1 -> Gain7/1
  Gain7/1 -> Integrator/1, [ax]
  [Velocity] -> Gain8/1
  Gain8/1 -> Tanh/1
  [Brake_pedal] -> G_Fbf/1
  [Velocity] -> Tanh_vx/1
  G_Fbf/1 -> P_Fbf/1
  Tanh_vx/1 -> P_Fbf/2
  P_Fbf/1 -> Sum/4

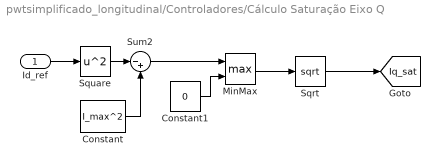
== system pwtsimplificado_longitudinal/Controladores/Cálculo Saturação Eixo Q ==
  Id_ref : Inport
  Constant : Constant  Value=I_max^2
  Constant1 : Constant  Value=0
  MinMax : MinMax  Function=max  Inputs=2
  Sqrt : Sqrt
  Square : Math  Operator=square
  Sum2 : Sum  Inputs=|-+
  tag scope: Iq_sat=global
  wires:
  Constant/1 -> Sum2/2
  Square/1 -> Sum2/1
  Id_ref/1 -> Square/1
  Sum2/1 -> MinMax/1
  Constant1/1 -> MinMax/2
  MinMax/1 -> Sqrt/1
  Sqrt/1 -> [Iq_sat]

== system pwtsimplificado_longitudinal/Controladores/Feed Forward eixo D ==
  FF_Vd : Scope
      settings: ActiveDisplayYMinimum=-29.823375414585424  ActiveDisplayYMaximum=39.827740751572378  DataLoggingMaxPoints=500000  DataLoggingVariableName=ScopeData9
  Gain3 : Gain  Gain=sigma
  Gain4 : Gain  Gain=Ls
  Product : Product
  We*Iqm*sigma*Ls : Outport
  tag scope: FF=global
  wires:
  Gain3/1 -> Gain4/1
  [Iqm] -> Product/2
  Product/1 -> Gain3/1
  [We] -> Product/1
  Gain4/1 -> [FF], FF_Vd/1, We*Iqm*sigma*Ls/1

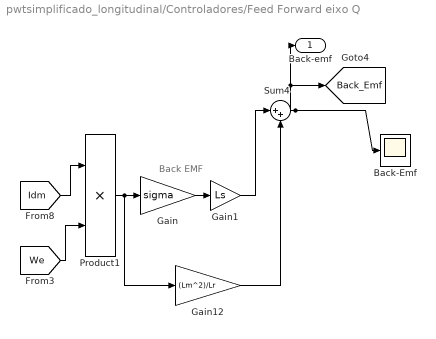
== system pwtsimplificado_longitudinal/Controladores/Feed Forward eixo Q ==
  note: Back EMF
  Back-Emf : Scope
      settings: ActiveDisplayYMinimum=-1218.68613  ActiveDisplayYMaximum=190.7559  DataLoggingMaxPoints=500000
  Gain : Gain  Gain=sigma
  Gain1 : Gain  Gain=Ls
  Gain12 : Gain  Gain=(Lm^2)/Lr
  Product1 : Product
  Sum4 : Sum  Inputs=|++
  Back-emf : Outport
  tag scope: Back_Emf=global
  wires:
  Gain/1 -> Gain1/1
  Gain12/1 -> Sum4/2
  [We] -> Product1/2
  Product1/1 -> Gain12/1, Gain/1
  Gain1/1 -> Sum4/1
  [Idm] -> Product1/1
  Sum4/1 -> Back-emf/1, [Back_Emf], Back-Emf/1

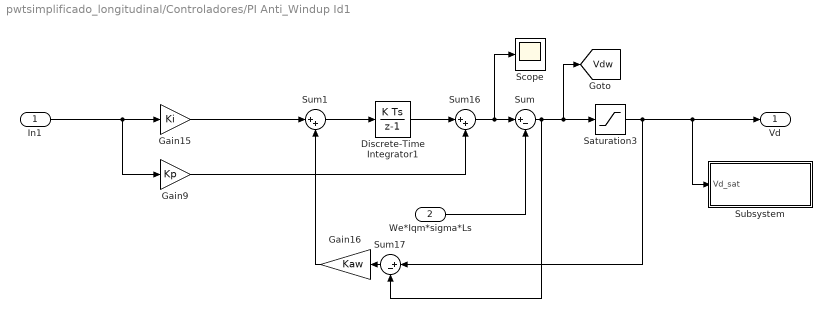
== system pwtsimplificado_longitudinal/Controladores/PI Anti_Windup Id1 ==
  In1 : Inport
  We*Iqm*sigma*Ls : Inport  Port=2
  Discrete-Time Integrator1 : DiscreteIntegrator  SampleTime=Amostragem  ICPrevOutput=DiscIntNeverNeededParam  ICPrevScaledInput=DiscIntNeverNeededParam
  Gain15 : Gain  Gain=Ki
  Gain16 : Gain  Gain=Kaw
  Gain9 : Gain  Gain=Kp
  Saturation3 : Saturate  UpperLimit=(Bv*Modulation_Target)/sqrt(3)  LowerLimit=-(Bv*Modulation_Target)/sqrt(3)
  Scope : Scope
      settings: ActiveDisplayYMinimum=1.3114775524509457  ActiveDisplayYMaximum=7.0252862645949152  DataLoggingVariableName=ScopeData15
  Subsystem : Subsystem
  Sum : Sum  Inputs=|+-
  Sum1 : Sum  Inputs=|++
  Sum16 : Sum  Inputs=|++
  Sum17 : Sum  Inputs=|+-
  Vd : Outport
  tag scope: Vdw=global
  wires:
  Sum1/1 -> Discrete-Time Integrator1/1
  Sum17/1 -> Gain16/1
  Gain9/1 -> Sum16/2
  Saturation3/1 -> Subsystem/1(Vd_sat), Vd/1, Sum17/1
  In1/1 -> Gain15/1, Gain9/1
  Sum16/1 -> Scope/1, Sum/1
  Sum/1 -> Sum17/2, [Vdw], Saturation3/1
  We*Iqm*sigma*Ls/1 -> Sum/2
  Gain15/1 -> Sum1/1
  Gain16/1 -> Sum1/2
  Discrete-Time Integrator1/1 -> Sum16/1

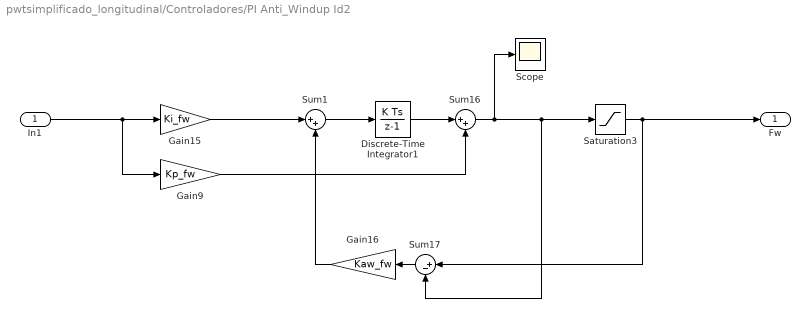
== system pwtsimplificado_longitudinal/Controladores/PI Anti_Windup Id2 ==
  In1 : Inport
  Discrete-Time Integrator1 : DiscreteIntegrator  SampleTime=Amostragem  ICPrevOutput=DiscIntNeverNeededParam  ICPrevScaledInput=DiscIntNeverNeededParam
  Gain15 : Gain  Gain=Ki_fw
  Gain16 : Gain  Gain=Kaw_fw
  Gain9 : Gain  Gain=Kp_fw
  Saturation3 : Saturate  UpperLimit=dImag_max  LowerLimit=dImag_min
  Scope : Scope
      settings: ActiveDisplayYMinimum=1.3114775524509457  ActiveDisplayYMaximum=7.0252862645949152  DataLoggingVariableName=ScopeData15
  Sum1 : Sum  Inputs=|++
  Sum16 : Sum  Inputs=|++
  Sum17 : Sum  Inputs=|+-
  Fw : Outport
  wires:
  Sum1/1 -> Discrete-Time Integrator1/1
  Sum17/1 -> Gain16/1
  Gain9/1 -> Sum16/2
  Saturation3/1 -> Fw/1, Sum17/1
  In1/1 -> Gain15/1, Gain9/1
  Sum16/1 -> Sum17/2, Saturation3/1, Scope/1
  Gain15/1 -> Sum1/1
  Gain16/1 -> Sum1/2
  Discrete-Time Integrator1/1 -> Sum16/1

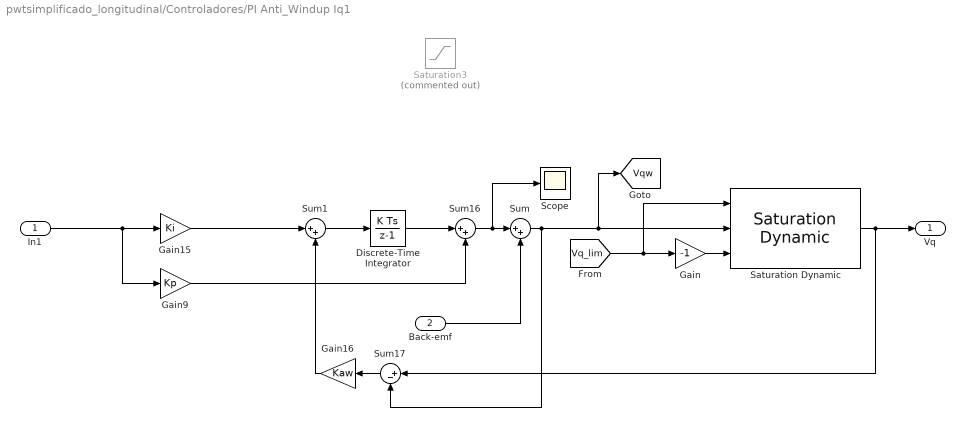
== system pwtsimplificado_longitudinal/Controladores/PI Anti_Windup Iq1 ==
  In1 : Inport
  Back-emf : Inport  Port=2
  Discrete-Time Integrator : DiscreteIntegrator  SampleTime=Amostragem  ICPrevOutput=DiscIntNeverNeededParam  ICPrevScaledInput=DiscIntNeverNeededParam
  Gain : Gain  Gain=-1
  Gain15 : Gain  Gain=Ki
  Gain16 : Gain  Gain=Kaw
  Gain9 : Gain  Gain=Kp
  Saturation Dynamic : simulink/Discontinuities/Saturation Dynamic  OutMin=[]  OutMax=[]  OutDataTypeStr=Inherit: Same as second input  OutDataType=fixdt(1, 16)  OutScaling=2^-10  DoSatur=off
  Saturation3 : Saturate  Commented=on  UpperLimit=Vq_lim  LowerLimit=-Vq_lim
  Scope : Scope
      settings: ActiveDisplayYMinimum=-1.055327868852459  ActiveDisplayYMaximum=3.944672131147541  DataLoggingVariableName=ScopeData14
  Sum : Sum  Inputs=|++
  Sum1 : Sum  Inputs=|++
  Sum16 : Sum  Inputs=|++
  Sum17 : Sum  Inputs=|+-
  Vq : Outport
  tag scope: Vqw=global
  wires:
  Sum1/1 -> Discrete-Time Integrator/1
  Sum17/1 -> Gain16/1
  Gain9/1 -> Sum16/2
  Saturation Dynamic/1 -> Vq/1, Sum17/1
  In1/1 -> Gain15/1, Gain9/1
  Sum16/1 -> Scope/1, Sum/1
  Sum/1 -> [Vqw], Saturation Dynamic/2, Sum17/2
  Back-emf/1 -> Sum/2
  Gain15/1 -> Sum1/1
  Gain16/1 -> Sum1/2
  Discrete-Time Integrator/1 -> Sum16/1
  Gain/1 -> Saturation Dynamic/3
  [Vq_lim] -> Saturation Dynamic/1, Gain/1

== system pwtsimplificado_longitudinal/Controladores/PI Anti_Windup Id1/Subsystem ==
  Vd_sat : Inport
  Constant : Constant  Value=Vmax^2
  Constant1 : Constant  Value=0
  MinMax : MinMax  Function=max  Inputs=2
  Sqrt : Sqrt
  Square : Math  Operator=square
  Sum2 : Sum  Inputs=|-+
  tag scope: Vq_lim=global
  wires:
  Constant/1 -> Sum2/2
  Square/1 -> Sum2/1
  Vd_sat/1 -> Square/1
  Sum2/1 -> MinMax/1
  Constant1/1 -> MinMax/2
  MinMax/1 -> Sqrt/1
  Sqrt/1 -> [Vq_lim]
